simulink model "robot_m3_test"  (R2024b)
settings: Solver=VariableStepAuto  StartTime=0.0  StopTime=2  MaxStep=0.01  RelTol=1e-3
PreLoadFcn:
  | % default test case 1 (all four joints move)
  | X_d = [150; 120; 250] / 1000;             % desired EE position, frame 0 (m)
  | V_d = [0.020; -0.010; 0.015];             % desired EE velocity (m/s)
  | if exist(fullfile(fileparts(get_param(bdroot,'FileName')),'..','Scripts'),'dir')
  |     addpath(fullfile(fileparts(get_param(bdroot,'FileName')),'..','Scripts'));
  | end
InitFcn:
  | % Milestone 03: call our MATLAB functions once (not inside the solver loop)
  | q_fun  = inverse_kinematics_func([0; -0.5; 1.0; -0.5], X_d);
  | qd_fun = inverse_velocity_kinematics(q_fun, V_d);
values from neighbouring files (symbols this model uses):
  X = T04(1:3, 4)    [forward_kinematics_func.m]    (also in inverse_jacobian_matrix.m = forward_kinematics_func())
undefined symbols (not defined in the file or in its folder): Y, Z
libraries: sm_lib x66, nesl_utility x14
(part 2 of 2)

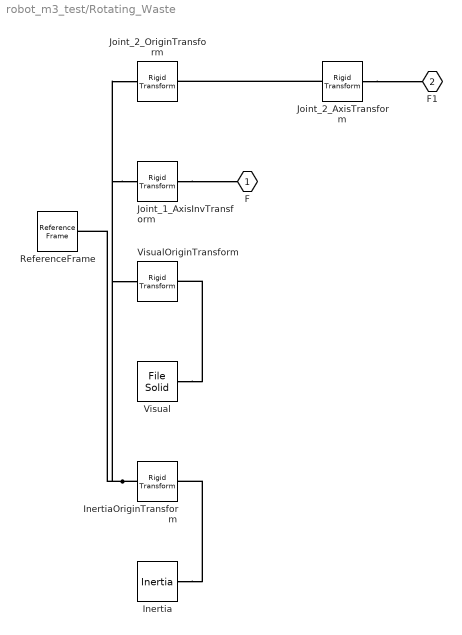
== system robot_m3_test/Rotating_Waste ==
  Inertia : sm_lib/Body Elements/Inertia  InertiaType=Custom  Mass=0.7  MassUnits=kg  CenterOfMass=[0, 0, 0]  CenterOfMassUnits=m  MomentsOfInertia=[0.0015, 0.0015, 0.0015]  MomentsOfInertiaUnits=kg*m^2  ProductsOfInertia=[0, 0, 0]  ProductsOfInertiaUnits=kg*m^2  GraphicType=None  MarkerShape=Inertia  MarkerSize=20  GraphicVisPropType=SimpleVisualProperties  GraphicDiffuseColor=[0.5 0.5 0.5]  GraphicOpacity=1  GraphicSpecularColor=[0.5 0.5 0.5 1.0]  GraphicAmbientColor=[0.15 0.15 0.15 1.0]  GraphicEmissiveColor=[0.0 0.0 0.0 1.0]  GraphicShininess=75
  InertiaOriginTransform : sm_lib/Frames and Transforms/Rigid Transform  RotationMethod=RotationSequence  FollAlignAxisA=+X  BaseAlignAxisA=+Y  FollAlignAxisB=+Y  BaseAlignAxisB=+Z  RotationStandardAxis=+Z  RotationAngle=0  RotationAngleUnits=deg  RotationArbitraryAxis=[0 0 1]  RotationSequenceAxes=BaseAxes  RotationSequence=XYZ  RotationSequenceAngles=[0, 0, 0]  RotationSequenceAnglesUnits=rad  RotationMatrix=[1 0 0;0 1 0;0 0 1]  Quaternion=[1 0 0 0]  TranslationMethod=Cartesian  TranslationCartesianOffset=[0, 0, 0]  TranslationCartesianOffsetUnits=m  TranslationStandardAxis=+Z  TranslationStandardOffset=0  TranslationStandardOffsetUnits=m  TranslationROffset=0  TranslationROffsetUnits=m  TranslationThetaOffset=0  TranslationThetaOffsetUnits=deg  TranslationZOffset=0  TranslationZOffsetUnits=m
  Joint_1_AxisInvTransform : sm_lib/Frames and Transforms/Rigid Transform  RotationMethod=ArbitraryAxis  FollAlignAxisA=+X  BaseAlignAxisA=+Y  FollAlignAxisB=+Y  BaseAlignAxisB=+Z  RotationStandardAxis=+Z  RotationAngle=0  RotationAngleUnits=rad  RotationArbitraryAxis=[1, 0, 0]  RotationSequenceAxes=FollowerAxes  RotationSequence=XYX  RotationSequenceAngles=[0 0 0]  RotationSequenceAnglesUnits=deg  RotationMatrix=[1 0 0;0 1 0;0 0 1]  Quaternion=[1 0 0 0]  TranslationMethod=Cartesian  TranslationCartesianOffset=[0, 0, 0]  TranslationCartesianOffsetUnits=m  TranslationStandardAxis=+Z  TranslationStandardOffset=0  TranslationStandardOffsetUnits=m  TranslationROffset=0  TranslationROffsetUnits=m  TranslationThetaOffset=0  TranslationThetaOffsetUnits=deg  TranslationZOffset=0  TranslationZOffsetUnits=m
  Joint_2_AxisTransform : sm_lib/Frames and Transforms/Rigid Transform  RotationMethod=ArbitraryAxis  FollAlignAxisA=+X  BaseAlignAxisA=+Y  FollAlignAxisB=+Y  BaseAlignAxisB=+Z  RotationStandardAxis=+Z  RotationAngle=0  RotationAngleUnits=rad  RotationArbitraryAxis=[1, 0, 0]  RotationSequenceAxes=FollowerAxes  RotationSequence=XYX  RotationSequenceAngles=[0 0 0]  RotationSequenceAnglesUnits=deg  RotationMatrix=[1 0 0;0 1 0;0 0 1]  Quaternion=[1 0 0 0]  TranslationMethod=Cartesian  TranslationCartesianOffset=[0, 0, 0]  TranslationCartesianOffsetUnits=m  TranslationStandardAxis=+Z  TranslationStandardOffset=0  TranslationStandardOffsetUnits=m  TranslationROffset=0  TranslationROffsetUnits=m  TranslationThetaOffset=0  TranslationThetaOffsetUnits=deg  TranslationZOffset=0  TranslationZOffsetUnits=m
  Joint_2_OriginTransform : sm_lib/Frames and Transforms/Rigid Transform  RotationMethod=RotationSequence  FollAlignAxisA=+X  BaseAlignAxisA=+Y  FollAlignAxisB=+Y  BaseAlignAxisB=+Z  RotationStandardAxis=+Z  RotationAngle=0  RotationAngleUnits=deg  RotationArbitraryAxis=[0 0 1]  RotationSequenceAxes=BaseAxes  RotationSequence=XYZ  RotationSequenceAngles=[1.5708, 0, 0]  RotationSequenceAnglesUnits=rad  RotationMatrix=[1 0 0;0 1 0;0 0 1]  Quaternion=[1 0 0 0]  TranslationMethod=Cartesian  TranslationCartesianOffset=[-2.7567e-05, 0.0061999, 0.04975]  TranslationCartesianOffsetUnits=m  TranslationStandardAxis=+Z  TranslationStandardOffset=0  TranslationStandardOffsetUnits=m  TranslationROffset=0  TranslationROffsetUnits=m  TranslationThetaOffset=0  TranslationThetaOffsetUnits=deg  TranslationZOffset=0  TranslationZOffsetUnits=m
  ReferenceFrame : sm_lib/Frames and Transforms/Reference Frame
  Visual : sm_lib/Body Elements/File Solid  ExtGeomFileName=meshes/Rotating_Waste.STL  UnitType=Custom  ExtGeomFileUnits=m  StepReaderType=HEX  ExportConvexHullGeometry=off  InertiaType=Custom  BasedOnType=DensityFromFile  Density=1000  DensityUnits=kg/m^3  Mass=0  MassUnits=kg  CenterOfMass=[0, 0, 0]  CenterOfMassUnits=m  MomentsOfInertia=[0, 0, 0]  MomentsOfInertiaUnits=kg*m^2  ProductsOfInertia=[0, 0, 0]  ProductsOfInertiaUnits=kg*m^2  GraphicType=FromGeometry  MarkerShape=Sphere  MarkerSize=10  GraphicVisPropType=SimpleVisualProperties  GraphicDiffuseColor=[0.7529400000000001, 0.7529400000000001, 0.7529400000000001]  GraphicOpacity=1  GraphicSpecularColor=[0.5 0.5 0.5 1.0]  GraphicAmbientColor=[0.15 0.15 0.15 1.0]  GraphicEmissiveColor=[0.0 0.0 0.0 1.0]  GraphicShininess=75  DoExposeReferenceFrame=on  SerializedFrames=<Frames/>
  VisualOriginTransform : sm_lib/Frames and Transforms/Rigid Transform  RotationMethod=RotationSequence  FollAlignAxisA=+X  BaseAlignAxisA=+Y  FollAlignAxisB=+Y  BaseAlignAxisB=+Z  RotationStandardAxis=+Z  RotationAngle=0  RotationAngleUnits=deg  RotationArbitraryAxis=[0 0 1]  RotationSequenceAxes=BaseAxes  RotationSequence=XYZ  RotationSequenceAngles=[0, 0, 0]  RotationSequenceAnglesUnits=rad  RotationMatrix=[1 0 0;0 1 0;0 0 1]  Quaternion=[1 0 0 0]  TranslationMethod=Cartesian  TranslationCartesianOffset=[0, 0, 0]  TranslationCartesianOffsetUnits=m  TranslationStandardAxis=+Z  TranslationStandardOffset=0  TranslationStandardOffsetUnits=m  TranslationROffset=0  TranslationROffsetUnits=m  TranslationThetaOffset=0  TranslationThetaOffsetUnits=deg  TranslationZOffset=0  TranslationZOffsetUnits=m
  F : PMIOPort  Side=Left
  F1 : PMIOPort  Port=2  Side=Right
  connections:
  Inertia/RConn1 -- InertiaOriginTransform/RConn1
  Joint_1_AxisInvTransform/RConn1 -- F/RConn1
  Joint_2_AxisTransform/RConn1 -- F1/RConn1
  Joint_2_AxisTransform/LConn1 -- Joint_2_OriginTransform/RConn1
  Joint_1_AxisInvTransform/LConn1 -- InertiaOriginTransform/LConn1 -- Joint_2_OriginTransform/LConn1 -- ReferenceFrame/RConn1 -- VisualOriginTransform/LConn1
  Visual/RConn1 -- VisualOriginTransform/RConn1

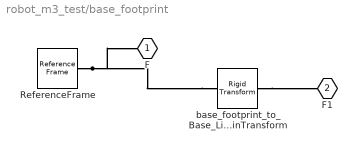
== system robot_m3_test/base_footprint ==
  ReferenceFrame : sm_lib/Frames and Transforms/Reference Frame
  base_footprint_to_Base_Link_OriginTransform : sm_lib/Frames and Transforms/Rigid Transform  RotationMethod=RotationSequence  FollAlignAxisA=+X  BaseAlignAxisA=+Y  FollAlignAxisB=+Y  BaseAlignAxisB=+Z  RotationStandardAxis=+Z  RotationAngle=0  RotationAngleUnits=deg  RotationArbitraryAxis=[0 0 1]  RotationSequenceAxes=BaseAxes  RotationSequence=XYZ  RotationSequenceAngles=[0, 0, 0]  RotationSequenceAnglesUnits=rad  RotationMatrix=[1 0 0;0 1 0;0 0 1]  Quaternion=[1 0 0 0]  TranslationMethod=Cartesian  TranslationCartesianOffset=[0, 0, 0.0438]  TranslationCartesianOffsetUnits=m  TranslationStandardAxis=+Z  TranslationStandardOffset=0  TranslationStandardOffsetUnits=m  TranslationROffset=0  TranslationROffsetUnits=m  TranslationThetaOffset=0  TranslationThetaOffsetUnits=deg  TranslationZOffset=0  TranslationZOffsetUnits=m
  F : PMIOPort  Side=Left
  F1 : PMIOPort  Port=2  Side=Right
  connections:
  base_footprint_to_Base_Link_OriginTransform/LConn1 -- ReferenceFrame/RConn1 -- F/RConn1
  base_footprint_to_Base_Link_OriginTransform/RConn1 -- F1/RConn1

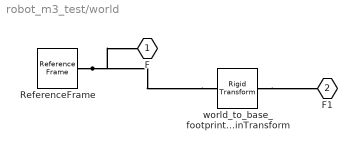
== system robot_m3_test/world ==
  ReferenceFrame : sm_lib/Frames and Transforms/Reference Frame
  world_to_base_footprint_OriginTransform : sm_lib/Frames and Transforms/Rigid Transform  RotationMethod=RotationSequence  FollAlignAxisA=+X  BaseAlignAxisA=+Y  FollAlignAxisB=+Y  BaseAlignAxisB=+Z  RotationStandardAxis=+Z  RotationAngle=0  RotationAngleUnits=deg  RotationArbitraryAxis=[0 0 1]  RotationSequenceAxes=BaseAxes  RotationSequence=XYZ  RotationSequenceAngles=[0, 0, 0]  RotationSequenceAnglesUnits=rad  RotationMatrix=[1 0 0;0 1 0;0 0 1]  Quaternion=[1 0 0 0]  TranslationMethod=Cartesian  TranslationCartesianOffset=[0, 0, 0]  TranslationCartesianOffsetUnits=m  TranslationStandardAxis=+Z  TranslationStandardOffset=0  TranslationStandardOffsetUnits=m  TranslationROffset=0  TranslationROffsetUnits=m  TranslationThetaOffset=0  TranslationThetaOffsetUnits=deg  TranslationZOffset=0  TranslationZOffsetUnits=m
  F : PMIOPort  Side=Left
  F1 : PMIOPort  Port=2  Side=Right
  connections:
  world_to_base_footprint_OriginTransform/LConn1 -- ReferenceFrame/RConn1 -- F/RConn1
  world_to_base_footprint_OriginTransform/RConn1 -- F1/RConn1

== matlab function robot_m3_test/Inverse Velocity Kinematics ==
  data: q1 input; qd1 output; q2 input; q3 input; q4 input; vx_d input; vy_d input; vz_d input; qd2 output; qd3 output; qd4 output
function [qd1, qd2, qd3, qd4] = ivk(q1, q2, q3, q4, vx_d, vy_d, vz_d)
% Inverse velocity kinematics, the same as inverse_velocity_kinematics:
%   q_dot = pinv(Jv(q)) * v      (Jv = linear part of the Jacobian, from the report)
psi3 = q2 - q3 + 0.012434;
psi4 = q2 - q3 + q4 - 0.069886;
rho  = 0.140*sin(q2) + 0.1329*sin(psi3) + 0.100245*sin(psi4);
rho2 = 0.140*cos(q2) + 0.1329*cos(psi3) + 0.100245*cos(psi4);
rho3 = -0.1329*cos(psi3) - 0.100245*cos(psi4);
rho4 = 0.100245*cos(psi4);
sig3 = 0.1329*sin(psi3) + 0.100245*sin(psi4);
s1 = sin(q1);
c1 = cos(q1);
Jv = [0.01226*c1 + rho*s1, -c1*rho2, -c1*rho3, -c1*rho4;
      0.01226*s1 - rho*c1, -s1*rho2, -s1*rho3, -s1*rho4;
      0,                   -rho,      sig3,     -0.100245*sin(psi4)];
qd = pinv(Jv) * [vx_d; vy_d; vz_d];
qd1 = qd(1);
qd2 = qd(2);
qd3 = qd(3);
qd4 = qd(4);

== matlab function robot_m3_test/Inverse Kinematics (Newton-Raphson) ==
  data: x_d input; q1 output; y_d input; z_d input; q2 output; q3 output; q4 output
function [q1, q2, q3, q4] = ik(x_d, y_d, z_d)
% Inverse position kinematics by Newton-Raphson, the same steps as inverse_kinematics_func:
%   q_new = q_old - pinv(dF/dq) * (FK(q_old) - X_d)
% FK and dF/dq are the closed-form equations of the report (frame 0, m, rad).
q = [0; -0.5; 1.0; -0.5];          % initial guess
Xd = [x_d; y_d; z_d];
for k = 1:100
    psi3 = q(2) - q(3) + 0.012434;
    psi4 = q(2) - q(3) + q(4) - 0.069886;
    rho  = 0.140*sin(q(2)) + 0.1329*sin(psi3) + 0.100245*sin(psi4);
    rho2 = 0.140*cos(q(2)) + 0.1329*cos(psi3) + 0.100245*cos(psi4);
    rho3 = -0.1329*cos(psi3) - 0.100245*cos(psi4);
    rho4 = 0.100245*cos(psi4);
    sig3 = 0.1329*sin(psi3) + 0.100245*sin(psi4);
    s1 = sin(q(1));
    c1 = cos(q(1));
    % forward kinematics
    X = [0.01226*s1 - rho*c1;
         -0.01226*c1 - rho*s1;
         0.04975 + 0.140*cos(q(2)) + 0.1329*cos(psi3) + 0.100245*cos(psi4)];
    F = X - Xd;
    if norm(F) < 1e-6
        break
    end
    % dF/dq (3x4) = linear part of the Jacobian
    Jv = [0.01226*c1 + rho*s1, -c1*rho2, -c1*rho3, -c1*rho4;
          0.01226*s1 - rho*c1, -s1*rho2, -s1*rho3, -s1*rho4;
          0,                   -rho,      sig3,     -0.100245*sin(psi4)];
    q = q - pinv(Jv) * F;
    q = mod(q + pi, 2*pi) - pi;    % keep angles in [-180, 180) deg
end
q1 = q(1);
q2 = q(2);
q3 = q(3);
q4 = q(4);

== matlab function robot_m3_test/Forward Kinematics ==
  data: x output; q1 input; y output; q2 input; q3 input; q4 input; z output
function [x, y, z] = fk(q1, q2, q3, q4)
% Forward position kinematics (Milestone 02), closed form from the report.
% Output in the WORLD frame (ground) to compare with Simscape: z + 0.0438 m.
psi3 = q2 - q3 + 0.012434;
psi4 = q2 - q3 + q4 - 0.069886;
rho = 0.140*sin(q2) + 0.1329*sin(psi3) + 0.100245*sin(psi4);
x = 0.01226*sin(q1) - rho*cos(q1);
y = -0.01226*cos(q1) - rho*sin(q1);
z = 0.04975 + 0.140*cos(q2) + 0.1329*cos(psi3) + 0.100245*cos(psi4) + 0.0438;

== matlab function robot_m3_test/Forward Velocity Kinematics ==
  data: q1 input; vx output; q2 input; q3 input; q4 input; qd1 input; qd2 input; qd3 input; qd4 input; vy output; vz output; wx output; wy output; wz output
function [vx, vy, vz, wx, wy, wz] = fvk(q1, q2, q3, q4, qd1, qd2, qd3, qd4)
% Forward velocity kinematics V_F = J(q) * q_dot, with the Jacobian of the report (m, rad).
psi3 = q2 - q3 + 0.012434;
psi4 = q2 - q3 + q4 - 0.069886;
rho  = 0.140*sin(q2) + 0.1329*sin(psi3) + 0.100245*sin(psi4);
rho2 = 0.140*cos(q2) + 0.1329*cos(psi3) + 0.100245*cos(psi4);
rho3 = -0.1329*cos(psi3) - 0.100245*cos(psi4);
rho4 = 0.100245*cos(psi4);
sig3 = 0.1329*sin(psi3) + 0.100245*sin(psi4);
s1 = sin(q1);
c1 = cos(q1);
vx = (0.01226*c1 + rho*s1)*qd1 - c1*rho2*qd2 - c1*rho3*qd3 - c1*rho4*qd4;
vy = (0.01226*s1 - rho*c1)*qd1 - s1*rho2*qd2 - s1*rho3*qd3 - s1*rho4*qd4;
vz = -rho*qd2 + sig3*qd3 - 0.100245*sin(psi4)*qd4;
wx = s1*(qd2 - qd3 + qd4);
wy = -c1*(qd2 - qd3 + qd4);
wz = qd1;
